simulink model "DCMotor"  (R2024b)
settings: Solver=VariableStepAuto  StartTime=0.0  StopTime=0.2  RelTol=1e-3
values from neighbouring files (symbols this model uses):
  b = J/tm    (= 0.000414117647059)    [param.m]
  Cr = 0    [param.m]
  EnableSaturation = 1    [param.m]
  J = 0.0000352    (= 3.52e-05)    [param.m]
  Km = 0.11    [param.m]
  Kpi = L/ti    (= 41)    [param.m]
  L = 0.0041    [param.m]
  R = 3.20    (= 3.2)    [param.m]
  Tii = L/R    (= 0.00128125)    [param.m]
  TSample = 0.0001    [param.m]
undefined symbols (not defined in the file or in its folder): dspblkCoreblockFVToolHelper, gcbh, Gmot, GmotInv, GmotInvz
settings Model: Creator=student  LastModifiedBy=student

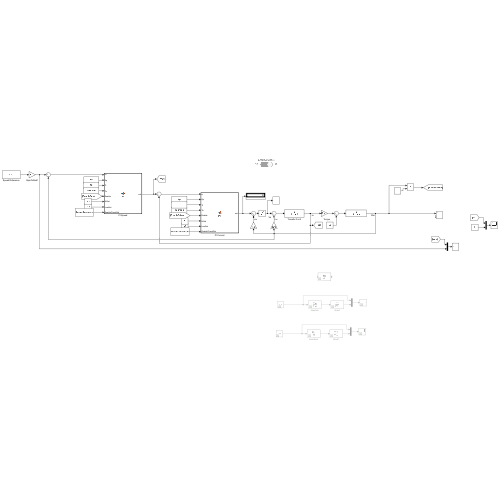
[thumbnail: Simulink's stored preview of the top-level diagram]
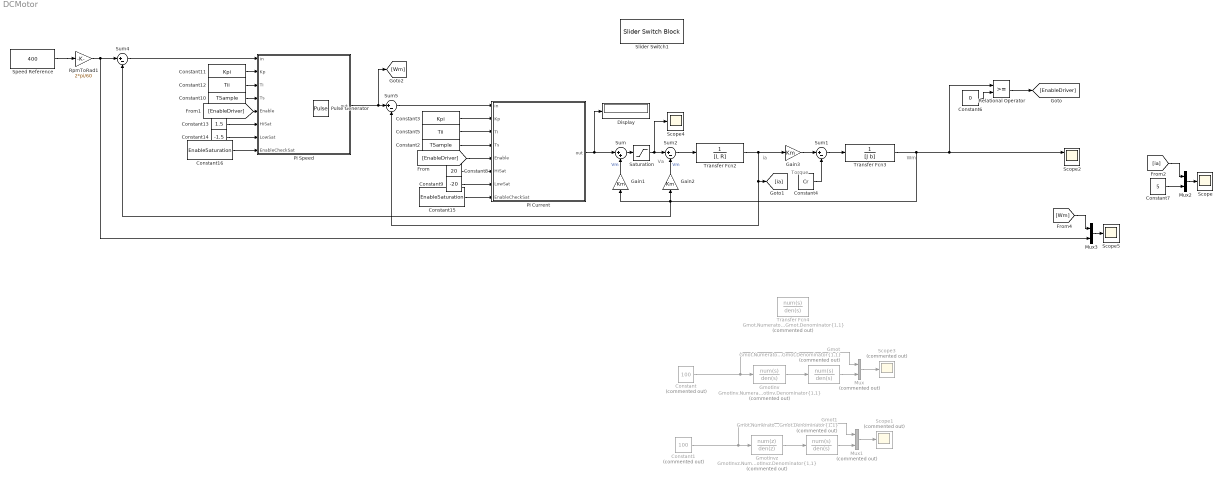
== system DCMotor ==
  note: Wm
  note: Torque
  note: Va
  note: ia
  Constant : Constant  Commented=on  Value=100
  Constant1 : Constant  Commented=on  Value=100
  Constant10 : Constant  Value=TSample  OutDataTypeStr=double
  Constant11 : Constant  Value=Kpi  OutDataTypeStr=double
  Constant12 : Constant  Value=Tii  OutDataTypeStr=double
  Constant13 : Constant  Value=1.5
  Constant14 : Constant  Value=-1.5
  Constant15 : Constant  Value=EnableSaturation  OutDataTypeStr=double
  Constant16 : Constant  Value=EnableSaturation  OutDataTypeStr=double
  Constant2 : Constant  Value=TSample  OutDataTypeStr=double
  Constant3 : Constant  Value=Kpi  OutDataTypeStr=double
  Constant4 : Constant  Value=Cr
  Constant5 : Constant  Value=Tii  OutDataTypeStr=double
  Constant6 : Constant  Value=0
  Constant7 : Constant  Value=5
  Constant8 : Constant  Value=20
  Constant9 : Constant  Value=-20
  Display : Display
  Gain1 : Gain  Gain=Km
  Gain2 : Gain  Gain=Km
  Gain3 : Gain  Gain=Km
  Gmot : TransferFcn  Commented=on  Numerator=Gmot.Numerator{1,1}  Denominator=Gmot.Denominator{1,1}
  Gmot1 : TransferFcn  Commented=on  Numerator=Gmot.Numerator{1,1}  Denominator=Gmot.Denominator{1,1}
  Gmotinv : TransferFcn  Commented=on  Numerator=GmotInv.Numerator{1,1}  Denominator=GmotInv.Denominator{1,1}
  Gmotinvz : DiscreteTransferFcn  Commented=on  LoadFcn=dspblkCoreblockFVToolHelper(gcbh,'load');  Numerator=GmotInvz.Numerator{1,1}  Denominator=GmotInvz.Denominator{1,1}
      settings: CopyFcn=dspblkCoreblockFVToolHelper(gcbh,'copy');  DeleteFcn=dspblkCoreblockFVToolHelper(gcbh,'close');  ModelCloseFcn=dspblkCoreblockFVToolHelper(gcbh,'close');  PreSaveFcn=dspblkCoreblockFVToolHelper(gcbh,'presave');  PostSaveFcn=dspblkCoreblockFVToolHelper(gcbh,'postsave');  CloseFcn=dspblkCoreblockFVToolHelper(gcbh,'close');
  Mux : Mux  Commented=on  Inputs=2
  Mux1 : Mux  Commented=on  Inputs=2
  Mux2 : Mux  Inputs=2
  Mux3 : Mux  Inputs=2
  PI Current : MATLAB Function  TreatAsAtomicUnit=on  SystemSampleTime=TSample
  PI Speed : MATLAB Function  TreatAsAtomicUnit=on  SystemSampleTime=TSample
  Pulse Generator : DiscretePulseGenerator  PulseType=Time based  Amplitude=5  Period=1  PulseWidth=50
  Relational Operator : RelationalOperator  OutDataTypeStr=boolean  RndMeth=Simplest  InputSameDT=off
  RpmToRad1 : Gain  Gain=2*pi/60
  Saturation : Saturate  UpperLimit=24  LowerLimit=-24
  Scope : Scope
  Scope1 : Scope  Commented=on
  Scope2 : Scope  NumInputPorts=2
  Scope3 : Scope  Commented=on
  Scope4 : Scope
  Scope5 : Scope
  Slider Switch1 : SliderSwitchBlock
      settings: Values={{'Off', 'On'}, [0 1]}
  Speed Reference : Constant  Value=400  OutDataTypeStr=double
  Sum : Sum  Inputs=|++
  Sum{1..2,4..5} (4 alike) : Sum  Inputs=|+-
  Transfer Fcn2 : TransferFcn  Denominator=[L R]
  Transfer Fcn3 : TransferFcn  Denominator=[J b]
  Transfer Fcn4 : TransferFcn  Commented=on  Numerator=Gmot.Numerator{1,1}  Denominator=Gmot.Denominator{1,1}
  wires:
  Sum2/1 -> Transfer Fcn2/1
  Transfer Fcn2/1 -> [ia], Sum5/2, Gain3/1
  Transfer Fcn3/1 -> Relational Operator/1, Scope2/1, Gain1/1, Gain2/1, Sum4/2
  Gain2/1 -> Sum2/2  "Vm"
  Gmotinv/1 -> Gmot/1
  Gmot/1 -> Mux/2
  Mux/1 -> Scope3/1
  Constant/1 -> Mux/1, Gmotinv/1
  Constant1/1 -> Gmotinvz/1, Mux1/1
  Mux1/1 -> Scope1/1
  Gmot1/1 -> Mux1/2
  Gmotinvz/1 -> Gmot1/1
  Gain3/1 -> Sum1/1
  Sum1/1 -> Transfer Fcn3/1
  Constant4/1 -> Sum1/2
  Gain1/1 -> Sum/2  "Vm"
  PI Current/1(out) -> Sum/1, Display/1
  Constant6/1 -> Relational Operator/2
  Relational Operator/1 -> [EnableDriver]
  [ia] -> Mux2/1
  Constant7/1 -> Mux2/2
  Mux2/1 -> Scope/1
  Sum/1 -> Saturation/1
  Saturation/1 -> Sum2/1, Scope4/1
  Constant16/1 -> PI Speed/8(EnableCheckSat)
  Constant14/1 -> PI Speed/7(LowSat)
  Constant13/1 -> PI Speed/6(HiSat)
  Constant12/1 -> PI Speed/3(Ti)
  Sum4/1 -> PI Speed/1(in)
  Constant11/1 -> PI Speed/2(Kp)
  Constant10/1 -> PI Speed/4(Ts)
  [EnableDriver] -> PI Speed/5(Enable)
  PI Speed/1(out) -> [Wm], Sum5/1
  Constant15/1 -> PI Current/8(EnableCheckSat)
  Sum5/1 -> PI Current/1(in)
  Constant5/1 -> PI Current/3(Ti)
  Constant8/1 -> PI Current/6(HiSat)
  Constant2/1 -> PI Current/4(Ts)
  Constant3/1 -> PI Current/2(Kp)
  Constant9/1 -> PI Current/7(LowSat)
  [EnableDriver] -> PI Current/5(Enable)
  Mux3/1 -> Scope5/1
  Speed Reference/1 -> RpmToRad1/1
  [Wm] -> Mux3/1
  RpmToRad1/1 -> Mux3/2, Sum4/1

== matlab function DCMotor/PI Speed ==
  data: in input; Kp input; Ti input; Ts input; out output; Enable input; HiSat input; LowSat input; EnableCheckSat input
function out = PI( in ,Kp , Ti , Ts , Enable, HiSat, LowSat, EnableCheckSat)
persistent in_prev out_prev 
% Initial Value
    if isempty( out_prev )
    out_prev = 0;
    end
    if isempty( in_prev )
    in_prev = 0;
    end
% G(s)=(Kp/Ti)*((1+Ti*s)/s) (Tustin)
% We run control only if motor is running
    if (Enable == 1)
    %I Calculate the output
     out = Kp*Ts/(2*Ti)*(in+in_prev) + Kp*(in-in_prev) + out_prev;
    else
    out = 0;
    in = 0;
    end
out_prev = out;
in_prev = in;

%saturazione provvisoria
out =25635;
if(EnableCheckSat == 1)
%check for saturation
if out > HiSat
out = HiSat;
elseif (out < LowSat)
out = LowSat; 
end
end
end

== matlab function DCMotor/PI Current ==
  data: in input; Kp input; Ti input; Ts input; out output; Enable input; HiSat input; LowSat input; EnableCheckSat input
function out = PI( in ,Kp , Ti , Ts , Enable, HiSat, LowSat, EnableCheckSat)
persistent in_prev out_prev 
% Initial Value
    if isempty( out_prev )
    out_prev = 0;
    end
    if isempty( in_prev )
    in_prev = 0;
    end
% G(s)=(Kp/Ti)*((1+Ti*s)/s) (Tustin)
% We run control only if motor is running
    if (Enable == 1)
    %I Calculate the output
     out = Kp*Ts/(2*Ti)*(in+in_prev) + Kp*(in-in_prev) + out_prev;
    else
    out = 0;
    in = 0;
    end
out_prev = out;
in_prev = in;

%saturazione provvisoria
out =25635;
if(EnableCheckSat == 1)
%check for saturation
if out > HiSat
out = HiSat;
elseif (out < LowSat)
out = LowSat; 
end
end
end
